simulink model "gauss_markov2"  (Simulink 9.1)
settings: Solver=ode45  StartTime=0.0  StopTime=10.0  RelTol=1e-3  EnableMultiTasking=on
values from neighbouring files (symbols this model uses):
  b = 0.1    [damposc.m]
undefined symbols (not defined in the file or in its folder): a
libraries: simulink x1
settings Model: Creator=1104070  LastModifiedBy=1104070
settings DataIOCC: LimitDataPoints=on  SignalLoggingSaveFormat=ModelDataLogs
settings OptimizationCC: BlockReduction=off  BooleanDataType=off  LifeSpan=auto
settings DebuggingCC: SaveWithParameterizedLinksMsg=none  SignalResolutionControl=TryResolveAllWithWarning  MultiTaskDSMMsg=warning  MultiTaskCondExecSysMsg=none  SFUnexpectedBacktrackingDiag=error  SFNoUnconditionalDefaultTransitionDiag=error  SFExecutionAtInitializationDiag=warning
settings HardwareCC: ProdBitPerPointer=64  ProdBitPerSizeT=64  ProdBitPerPtrDiffT=64  ProdLargestAtomicFloat=Float  ProdIntDivRoundTo=Zero  ProdEndianess=LittleEndian  ProdWordSize=64  ProdHWDeviceType=Intel->x86-64 (Windows64)  TargetUnknown=on
settings CodeAppCC: StateflowObjectComments=off
settings ConfigComp: CovMetricSettings=dwe

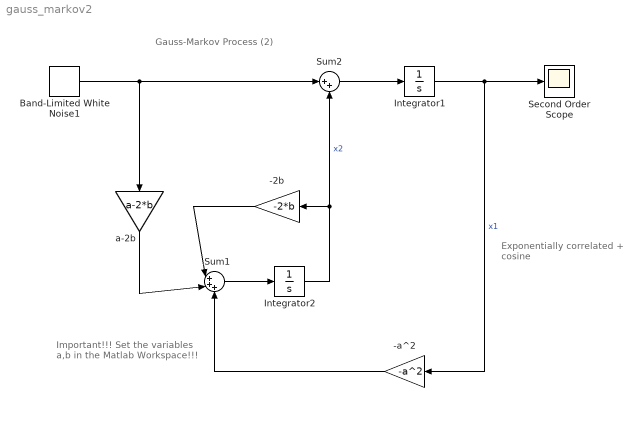
== system gauss_markov2 ==
  note: Important!!!
      | Set the variables a,b in the
      | Matlab Workspace!!!
  note: Exponentially correlated +
      | cosine
  note: Gauss-Markov Process (2)
  -2b : Gain  Gain=-2*b  SaturateOnIntegerOverflow=on  OutDataTypeStr=Inherit: Same as input  ParamDataTypeStr=Inherit: Same as input
  -a^2 : Gain  Gain=-a^2  SaturateOnIntegerOverflow=on  OutDataTypeStr=Inherit: Same as input  ParamDataTypeStr=Inherit: Same as input
  Band-Limited White Noise1 : simulink/Sources/Band-Limited White Noise  Cov=[10]  Ts=0.01  seed=[23341]
  Integrator1 : Integrator
  Integrator2 : Integrator
  Second Order Scope : Scope
  Sum1 : Sum  Inputs=|+++  SaturateOnIntegerOverflow=on  InputSameDT=on  OutDataTypeStr=Inherit: Same as first input
  Sum2 : Sum  Inputs=|++  SaturateOnIntegerOverflow=on  InputSameDT=on  OutDataTypeStr=Inherit: Same as first input
  a-2b : Gain  Gain=a-2*b  SaturateOnIntegerOverflow=on  OutDataTypeStr=Inherit: Same as input  ParamDataTypeStr=Inherit: Same as input
  wires:
  Integrator1/1 -> Second Order Scope/1, -a^2/1  "x1"
  Band-Limited White Noise1/1 -> Sum2/1, a-2b/1
  Integrator2/1 -> -2b/1, Sum2/2  "x2"
  -2b/1 -> Sum1/1
  a-2b/1 -> Sum1/2
  Sum1/1 -> Integrator2/1
  -a^2/1 -> Sum1/3
  Sum2/1 -> Integrator1/1
